simulink model "Logical_Architecture"  (R2025b)
settings: Solver=VariableStepAuto  StartTime=0.0  StopTime=10.0  RelTol=1e-3
settings Model: Creator=prati  LastModifiedBy=prati

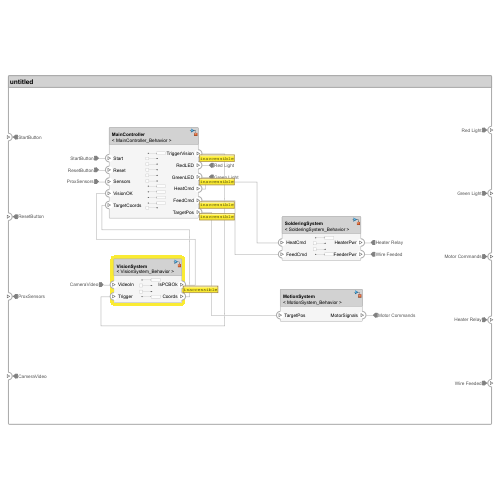
[thumbnail: Simulink's stored preview of the top-level diagram]
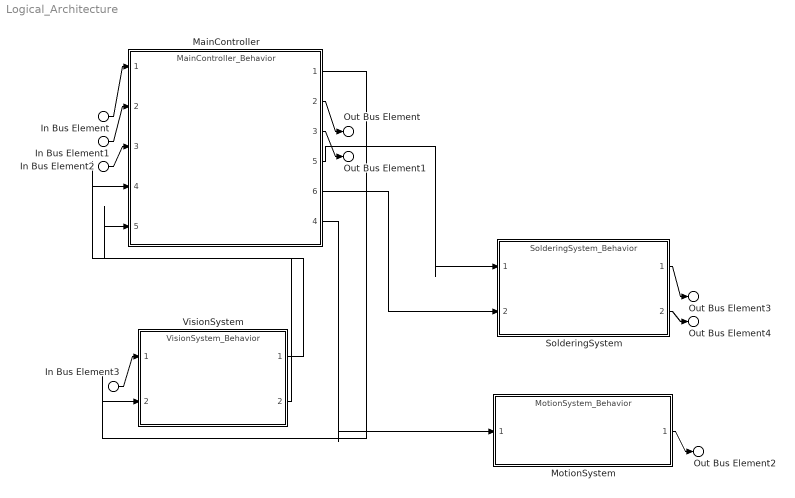
== system Logical_Architecture ==
  In Bus Element : Inport  PortName=StartButton
  In Bus Element1 : Inport  Port=2  PortName=ResetButton
  In Bus Element2 : Inport  Port=3  PortName=ProxSensors
  In Bus Element3 : Inport  Port=4  PortName=CameraVideo
  MainController : ModelReference  ModelNameDialog=MainController_Behavior  SimulationMode=Normal  ModelReferenceVersion=1.2
      settings: PortSchema="{\"entries\":[{\"content\":{\"headerSize\":38,\"margin\":15,\"minimumSpacing\":25,\"sides\":[{\"content\":{\"connectorIds\":[\"In1\",\"In2\",\"In3\",\"In4\",\"In5\"]},\"type\":\"ConnectorPlacement.EquallySpacedRectSide\",\"uuid\":\"49210b06-30c6-44db-9126-af21fea4dbd6\"},{\"content\":{\"connectorIds\":[\"Out1\",\"Out2\",\"Out3\",\"Out5\",\"Out6\",\"Out4\"],\"side\":\"RIGHT\"},\"type\":\"ConnectorPlacement.EquallySpacedRectSide\",\"uuid\":\"5290e3af-7623-45d1-a5f1-09aa0f6ad954\"},{\"content\":{\"side\":\"TOP\"},\"type\":\"ConnectorPlacement.EquallySpacedRectSide\",\"uuid\":\"561726a7-11cd-4b1d-b814-c780a569f7ed\"}]},\"type\":\"ConnectorPlacement.EquallySpacedConnector\",\"uuid\":\"30243aa0-d27d-4e18-8d36-bb20012f9122\"}],\"packageUris\":[\"http://schema.mathworks.com/mf0/Connector/R2020b\"],\"version\":\"1.0\"}"
  MotionSystem : ModelReference  ModelNameDialog=MotionSystem_Behavior  SimulationMode=Normal  ModelReferenceVersion=1.2
      settings: PortSchema="{\"entries\":[{\"content\":{\"headerSize\":38,\"margin\":15,\"minimumSpacing\":25,\"sides\":[{\"content\":{\"connectorIds\":[\"In1\"]},\"type\":\"ConnectorPlacement.EquallySpacedRectSide\",\"uuid\":\"49210b06-30c6-44db-9126-af21fea4dbd6\"},{\"content\":{\"connectorIds\":[\"Out1\"],\"side\":\"RIGHT\"},\"type\":\"ConnectorPlacement.EquallySpacedRectSide\",\"uuid\":\"5290e3af-7623-45d1-a5f1-09aa0f6ad954\"},{\"content\":{\"side\":\"TOP\"},\"type\":\"ConnectorPlacement.EquallySpacedRectSide\",\"uuid\":\"561726a7-11cd-4b1d-b814-c780a569f7ed\"}]},\"type\":\"ConnectorPlacement.EquallySpacedConnector\",\"uuid\":\"30243aa0-d27d-4e18-8d36-bb20012f9122\"}],\"packageUris\":[\"http://schema.mathworks.com/mf0/Connector/R2020b\"],\"version\":\"1.0\"}"
  SolderingSystem : ModelReference  ModelNameDialog=SolderingSystem_Behavior  SimulationMode=Normal  ModelReferenceVersion=1.2
      settings: PortSchema="{\"entries\":[{\"content\":{\"headerSize\":38,\"margin\":15,\"minimumSpacing\":25,\"sides\":[{\"content\":{\"connectorIds\":[\"In1\",\"In2\"]},\"type\":\"ConnectorPlacement.EquallySpacedRectSide\",\"uuid\":\"49210b06-30c6-44db-9126-af21fea4dbd6\"},{\"content\":{\"connectorIds\":[\"Out1\",\"Out2\"],\"side\":\"RIGHT\"},\"type\":\"ConnectorPlacement.EquallySpacedRectSide\",\"uuid\":\"5290e3af-7623-45d1-a5f1-09aa0f6ad954\"},{\"content\":{\"side\":\"TOP\"},\"type\":\"ConnectorPlacement.EquallySpacedRectSide\",\"uuid\":\"561726a7-11cd-4b1d-b814-c780a569f7ed\"}]},\"type\":\"ConnectorPlacement.EquallySpacedConnector\",\"uuid\":\"30243aa0-d27d-4e18-8d36-bb20012f9122\"}],\"packageUris\":[\"http://schema.mathworks.com/mf0/Connector/R2020b\"],\"version\":\"1.0\"}"
  VisionSystem : ModelReference  ModelNameDialog=VisionSystem_Behavior  SimulationMode=Normal  ModelReferenceVersion=1.2
      settings: PortSchema="{\"entries\":[{\"content\":{\"headerSize\":38,\"margin\":15,\"minimumSpacing\":25,\"sides\":[{\"content\":{\"connectorIds\":[\"In1\",\"In2\"]},\"type\":\"ConnectorPlacement.EquallySpacedRectSide\",\"uuid\":\"49210b06-30c6-44db-9126-af21fea4dbd6\"},{\"content\":{\"connectorIds\":[\"Out1\",\"Out2\"],\"side\":\"RIGHT\"},\"type\":\"ConnectorPlacement.EquallySpacedRectSide\",\"uuid\":\"5290e3af-7623-45d1-a5f1-09aa0f6ad954\"},{\"content\":{\"side\":\"TOP\"},\"type\":\"ConnectorPlacement.EquallySpacedRectSide\",\"uuid\":\"561726a7-11cd-4b1d-b814-c780a569f7ed\"}]},\"type\":\"ConnectorPlacement.EquallySpacedConnector\",\"uuid\":\"30243aa0-d27d-4e18-8d36-bb20012f9122\"}],\"packageUris\":[\"http://schema.mathworks.com/mf0/Connector/R2020b\"],\"version\":\"1.0\"}"
  Out Bus Element : Outport  PortName=Red Light
  Out Bus Element1 : Outport  Port=2  PortName=Green Light
  Out Bus Element2 : Outport  Port=3  PortName=Motor Commands
  Out Bus Element3 : Outport  Port=4  PortName=Heater Relay
  Out Bus Element4 : Outport  Port=5  PortName=Wire Feeded
  wires:
  In Bus Element/1 -> MainController/1
  In Bus Element1/1 -> MainController/2
  In Bus Element2/1 -> MainController/3
  In Bus Element3/1 -> VisionSystem/1
  SolderingSystem/1 -> Out Bus Element3/1
  SolderingSystem/2 -> Out Bus Element4/1
  MotionSystem/1 -> Out Bus Element2/1
  MainController/2 -> Out Bus Element/1
  MainController/3 -> Out Bus Element1/1
  MainController/4 -> MotionSystem/1
  MainController/1 -> VisionSystem/2
  MainController/5 -> SolderingSystem/1
  MainController/6 -> SolderingSystem/2
  VisionSystem/1 -> MainController/4
  VisionSystem/2 -> MainController/5
